simulink model "Adaptive"  (R2022b)
settings: Solver=VariableStepAuto  StartTime=0.0  StopTime=50  RelTol=1e-3
libraries: simulink x1
settings Model: Creator=ali14  LastModifiedBy=ali14

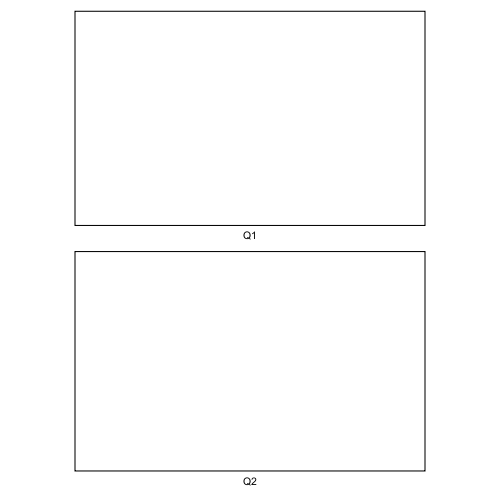
[thumbnail: Simulink's stored preview of the top-level diagram]
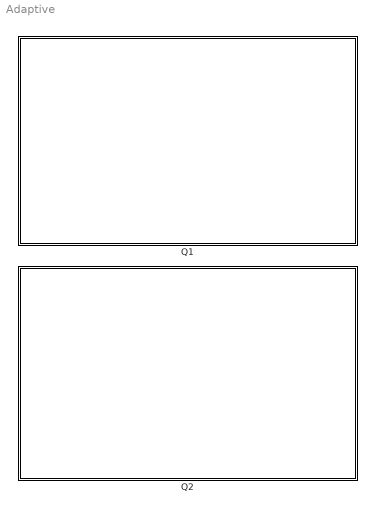
== system Adaptive ==
  Q1 : Subsystem
  Q2 : Subsystem

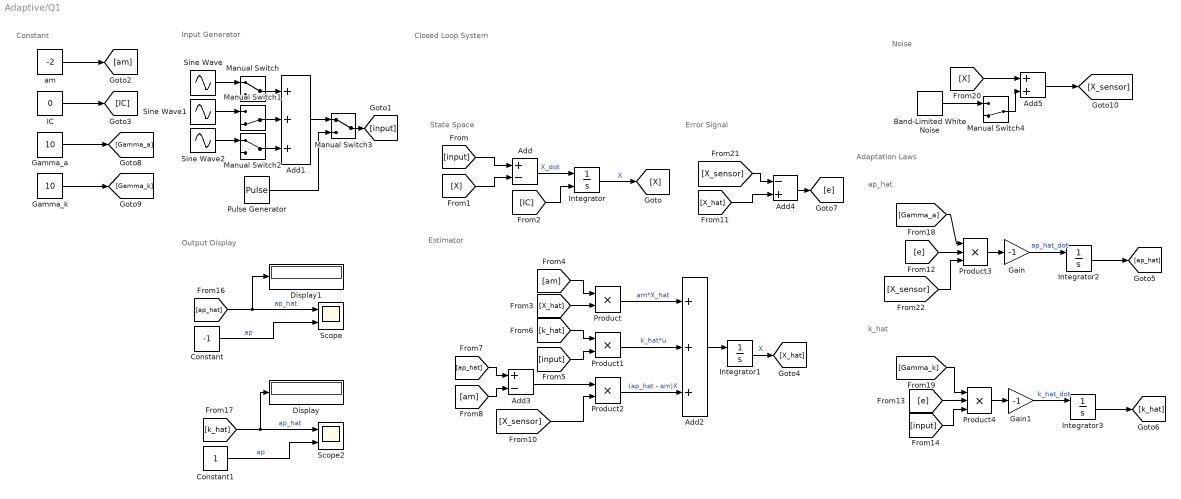
== system Adaptive/Q1 ==
  note: Noise
  note: Closed Loop System
  note: Estimator
  note: Error Signal
  note: Output Display
  note: ap_hat
  note: Adaptation Laws
  note: State Space
  note: Constant
  note: Input Generator
  note: k_hat
  Add : Sum  Inputs=+-
  Add1 : Sum  Inputs=+++
  Add2 : Sum  Inputs=+++
  Add3 : Sum  Inputs=+-
  Add4 : Sum  Inputs=-+
  Add5 : Sum
  Band-Limited White Noise : simulink/Sources/Band-Limited White Noise  Cov=[0.001]  Ts=0.1  seed=[23341]
  Constant : Constant  Value=-1
  Constant1 : Constant
  Display : Display
  Display1 : Display
  Gain : Gain  Gain=-1
  Gain1 : Gain  Gain=-1
  Gamma_a : Constant  Value=10
  Gamma_k : Constant  Value=10
  IC : Constant  Value=0
  Integrator{,1..3} (4 alike) : Integrator  InitialConditionSource=external
  Manual Switch : ManualSwitch
  Manual Switch1 : ManualSwitch  CurrentSetting=0
  Manual Switch2 : ManualSwitch
  Manual Switch3 : ManualSwitch
  Manual Switch4 : ManualSwitch  CurrentSetting=0
  Product : Product
  Product1 : Product
  Product2 : Product
  Product3 : Product  Inputs=3
  Product4 : Product  Inputs=3
  Pulse Generator : DiscretePulseGenerator  PulseType=Time based  Amplitude=5  Period=1  PulseWidth=50
  Scope : Scope  NumInputPorts=2
  Scope2 : Scope  NumInputPorts=2
  Sine Wave : Sin  SampleTime=0
  Sine Wave1 : Sin  Frequency=2  SampleTime=0
  Sine Wave2 : Sin  Frequency=3  SampleTime=0
  am : Constant  Value=-2
  wires:
  Add/1 -> Integrator/1  "X_dot"
  [input] -> Add/1
  Integrator/1 -> [X]  "X"
  [X] -> Add/2
  Manual Switch/1 -> Add1/1
  Sine Wave/1 -> Manual Switch/1
  Manual Switch1/1 -> Add1/2
  Manual Switch2/1 -> Add1/3
  Sine Wave1/1 -> Manual Switch1/1
  Sine Wave2/1 -> Manual Switch2/1
  am/1 -> [am]
  IC/1 -> [IC]
  [IC] -> Integrator/2
  Add2/1 -> Integrator1/1
  Integrator1/1 -> [X_hat]  "X"
  [X_hat] -> Product/2
  [am] -> Product/1
  Product/1 -> Add2/1  "am*X_hat"
  Product1/1 -> Add2/2  "k_hat*u"
  [input] -> Product1/2
  [k_hat] -> Product1/1
  Product2/1 -> Add2/3  "(ap_hat - am)X"
  Add3/1 -> Product2/1
  [ap_hat] -> Add3/1
  [am] -> Add3/2
  [X_sensor] -> Product2/2
  Integrator2/1 -> [ap_hat]
  Integrator3/1 -> [k_hat]
  [X_sensor] -> Add4/1
  [X_hat] -> Add4/2
  Add4/1 -> [e]
  Product3/1 -> Gain/1
  Gain/1 -> Integrator2/1  "ap_hat_dot"
  Product4/1 -> Gain1/1
  Gain1/1 -> Integrator3/1  "k_hat_dot"
  [ap_hat] -> Display1/1, Scope/1  "ap_hat"
  Constant/1 -> Scope/2  "ap"
  Constant1/1 -> Scope2/2  "ap"
  [k_hat] -> Display/1, Scope2/1  "ap_hat"
  [X_sensor] -> Product3/3
  [e] -> Product3/2
  [input] -> Product4/3
  [e] -> Product4/2
  Gamma_a/1 -> [Gamma_a]
  Gamma_k/1 -> [Gamma_k]
  [Gamma_a] -> Product3/1
  [Gamma_k] -> Product4/1
  Pulse Generator/1 -> Manual Switch3/2
  Add1/1 -> Manual Switch3/1
  Manual Switch3/1 -> [input]
  [X] -> Add5/1
  Manual Switch4/1 -> Add5/2
  Band-Limited White Noise/1 -> Manual Switch4/1
  Add5/1 -> [X_sensor]

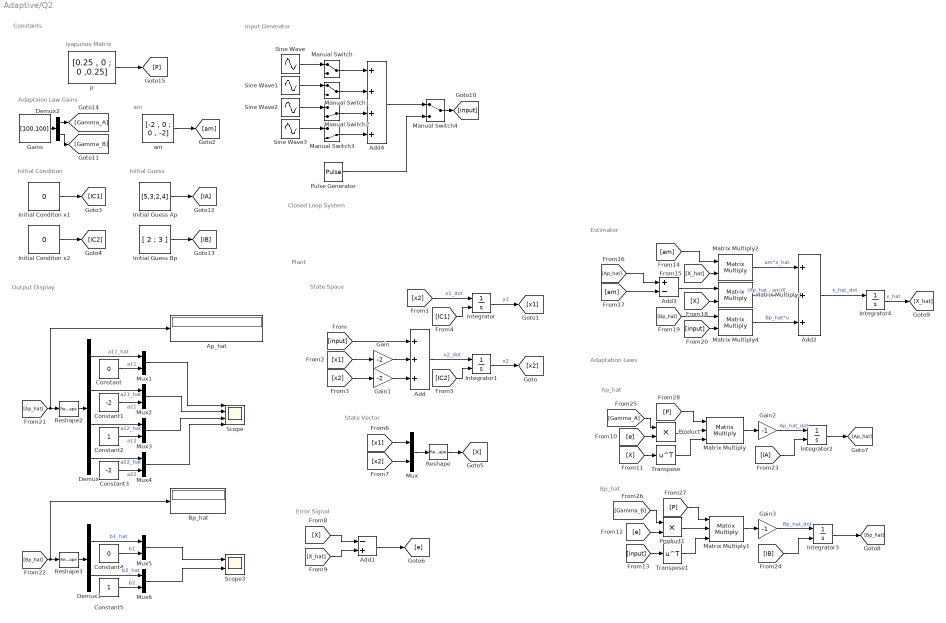
== system Adaptive/Q2 ==
  note: Closed Loop System
  note: Plant
  note: am
  note: Initial Condition
  note: Bp_hat
  note: Output Display
  note: Estimator
  note: Input Generator
  note: State Vector
  note: Error Signal
  note: State Space
  note: Constants
  note: Ap_hat
  note: Adaptation Laws
  note: Initial Guess
  note: Adaptaion Law Gains
  note: lyapunov Matrix
  Add : Sum  Inputs=+++
  Add1 : Sum  Inputs=-+
  Add2 : Sum  Inputs=+++
  Add3 : Sum  Inputs=+-
  Add4 : Sum  Inputs=++++
  Ap_hat : Display
  Bp_hat : Display
  Constant : Constant  Value=0
  Constant1 : Constant  Value=-2
  Constant2 : Constant
  Constant3 : Constant  Value=-2
  Constant4 : Constant  Value=0
  Constant5 : Constant
  Demux : Demux
  Demux1 : Demux  Outputs=2
  Demux2 : Demux  Outputs=2
  Gain : Gain  Gain=-2
  Gain1 : Gain  Gain=-2
  Gain2 : Gain  Gain=-1
  Gain3 : Gain  Gain=-1
  Gains : Constant  Value=[100,100]
  Initial Conditon x1 : Constant  Value=0
  Initial Conditon x2 : Constant  Value=0
  Initial Guess Ap : Constant  Value=[5,3;2,4]  VectorParams1D=off
  Initial Guess Bp : Constant  Value=[ 2 ; 3 ]  VectorParams1D=off
  Integrator{,1..4} (5 alike) : Integrator  InitialConditionSource=external
  Manual Switch : ManualSwitch
  Manual Switch1 : ManualSwitch
  Manual Switch2 : ManualSwitch  CurrentSetting=0
  Manual Switch3 : ManualSwitch  CurrentSetting=0
  Manual Switch4 : ManualSwitch
  Matrix Multiply : Product  Inputs=3  Multiplication=Matrix(*)
  Matrix Multiply1 : Product  Inputs=3  Multiplication=Matrix(*)
  Matrix Multiply2 : Product  Multiplication=Matrix(*)
  Matrix Multiply3 : Product  Multiplication=Matrix(*)
  Matrix Multiply4 : Product  Multiplication=Matrix(*)
  Mux{,1..6} (7 alike) : Mux  Inputs=2
  Product : Product
  Product1 : Product
  Pulse Generator : DiscretePulseGenerator  PulseType=Time based  Amplitude=5  Period=1  PulseWidth=50
  Reshape : Reshape  OutputDimensionality=Column vector (2-D)
  Reshape2 : Reshape  OutputDimensionality=Column vector (2-D)
  Reshape3 : Reshape  OutputDimensionality=Column vector (2-D)
  Scope : Scope  NumInputPorts=4
  Scope3 : Scope  NumInputPorts=2
  Sine Wave : Sin  SampleTime=0
  Sine Wave1 : Sin  Frequency=2  SampleTime=0
  Sine Wave2 : Sin  Frequency=3  SampleTime=0
  Sine Wave3 : Sin  Frequency=4  SampleTime=0
  Transpose : Math  Operator=transpose
  Transpose1 : Math  Operator=transpose
  am : Constant  Value=[-2 , 0 ; 0 , -2]
  p : Constant  Value=[0.25 , 0 ; 0 ,0.25]
  wires:
  am/1 -> [am]
  Sine Wave2/1 -> Manual Switch2/1
  Mux2/1 -> Scope/2
  [IC1] -> Integrator/2
  Initial Conditon x2/1 -> [IC2]
  Integrator1/1 -> [x2]  "x2"
  Constant4/1 -> Mux5/2  "b1"
  Mux1/1 -> Scope/1
  [x2] -> Gain1/1
  Sine Wave3/1 -> Manual Switch3/1
  [Ap_hat] -> Ap_hat/1, Reshape2/1
  [Bp_hat] -> Matrix Multiply4/1
  [x2] -> Mux/2
  [x2] -> Integrator/1  "x1_dot"
  Integrator3/1 -> [Bp_hat]
  [input] -> Add/1
  Reshape/1 -> [X]
  [X] -> Transpose/1
  Matrix Multiply3/1 -> Add2/2  "(Ap_hat - am)X"
  [X_hat] -> Add1/2
  Mux4/1 -> Scope/4
  Gain/1 -> Add/2
  Mux/1 -> Reshape/1
  Initial Guess Bp/1 -> [IB]
  Matrix Multiply/1 -> Gain2/1
  Add/1 -> Integrator1/1  "x2_dot"
  Constant5/1 -> Mux6/2  "b2"
  Matrix Multiply4/1 -> Add2/3  "Bp_hat*u"
  Integrator2/1 -> [Ap_hat]
  Demux/4 -> Mux4/1  "a22_hat"
  Sine Wave1/1 -> Manual Switch1/1
  [am] -> Matrix Multiply2/1
  Initial Guess Ap/1 -> [IA]
  [e] -> Product1/2
  [X] -> Add1/1
  Initial Conditon x1/1 -> [IC1]
  [am] -> Add3/2
  [Ap_hat] -> Add3/1
  Add2/1 -> Integrator4/1  "x_hat_dot"
  Demux1/2 -> Mux6/1  "b2_hat"
  Matrix Multiply2/1 -> Add2/1  "am*x_hat"
  Demux/3 -> Mux3/1  "a12_hat"
  Manual Switch2/1 -> Add4/3
  [input] -> Matrix Multiply4/2
  Add1/1 -> [e]
  [Gamma_A] -> Product/1
  Integrator4/1 -> [X_hat]  "x_hat"
  Gain3/1 -> Integrator3/1  "Bp_hat_dot"
  Gain2/1 -> Integrator2/1  "Ap_hat_dot"
  Gain1/1 -> Add/3
  Constant3/1 -> Mux4/2  "a22"
  Mux3/1 -> Scope/3
  Constant2/1 -> Mux3/2  "a12"
  Demux/2 -> Mux2/1  "a21_hat"
  Sine Wave/1 -> Manual Switch/1
  Transpose1/1 -> Matrix Multiply1/3
  Reshape2/1 -> Demux/1
  Constant/1 -> Mux1/2  "a11"
  Manual Switch3/1 -> Add4/4
  Constant1/1 -> Mux2/2  "a21"
  [x1] -> Mux/1
  Add3/1 -> Matrix Multiply3/1
  Matrix Multiply1/1 -> Gain3/1
  Mux6/1 -> Scope3/2
  Product1/1 -> Matrix Multiply1/2
  [IA] -> Integrator2/2
  Demux/1 -> Mux1/1  "a11_hat"
  Integrator/1 -> [x1]  "x1"
  Mux5/1 -> Scope3/1
  Demux1/1 -> Mux5/1  "b1_hat"
  Manual Switch/1 -> Add4/1
  p/1 -> [P]
  Demux2/2 -> [Gamma_B]
  [X] -> Matrix Multiply3/2
  [IB] -> Integrator3/2
  [IC2] -> Integrator1/2
  [Gamma_B] -> Product1/1
  [X_hat] -> Matrix Multiply2/2
  [Bp_hat] -> Bp_hat/1, Reshape3/1
  [x1] -> Gain/1
  Gains/1 -> Demux2/1
  Demux2/1 -> [Gamma_A]
  [input] -> Transpose1/1
  Product/1 -> Matrix Multiply/2
  Manual Switch1/1 -> Add4/2
  [e] -> Product/2
  [P] -> Matrix Multiply/1
  [P] -> Matrix Multiply1/1
  Transpose/1 -> Matrix Multiply/3
  Reshape3/1 -> Demux1/1
  Manual Switch4/1 -> [input]
  Add4/1 -> Manual Switch4/1
  Pulse Generator/1 -> Manual Switch4/2
